simulink model "Kapitsa0x2Dpendulum"  (R2023b)
settings: Solver=VariableStepAuto  StartTime=0.0  StopTime=10  MaxStep=0.05  RelTol=1e-3
values from neighbouring files (symbols this model uses):
  Freq = freq_m(i)    [untitled.m]
  i = m*l^2    [mask1.m]
libraries: simulink_extras x2
settings Model: Creator=macbook  LastModifiedBy=macbook
settings DataIOCC: ReturnWorkspaceOutputs=off

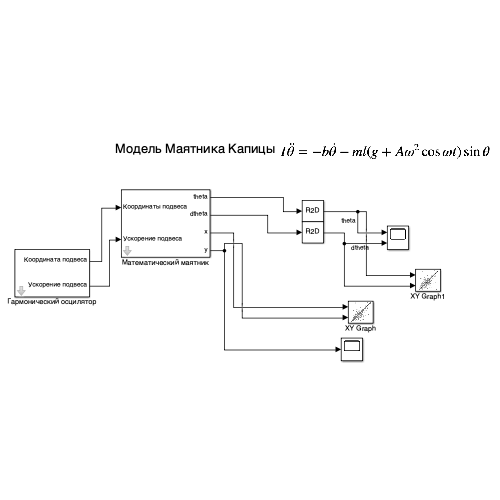
[thumbnail: Simulink's stored preview of the top-level diagram]
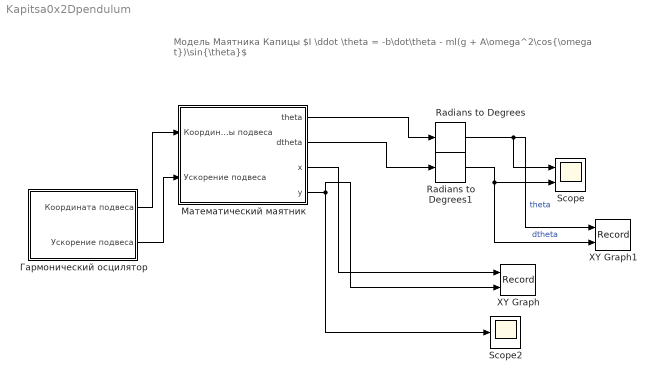
== system Kapitsa0x2Dpendulum ==
  note: Модель Маятника Капицы $I \ddot \theta = -b\dot\theta - ml(g + A\omega^2\cos{\omega t})\sin{\theta}$
  Radians to Degrees : simulink_extras/Transformations/Radians to Degrees
  Radians to Degrees1 : simulink_extras/Transformations/Radians to Degrees
  Scope : Scope  NumInputPorts=2
  Scope2 : Scope
  XY Graph : Record  FileSettingsInternal="{\"entries\":[{\"content\":{\"excelSettings\":{\"content\":{},\"type\":\"Streamout.ExcelSettings\"}},\"type\":\"Streamout.FileSettingStorage\",\"uuid\":\"\"}],\"packageUris\":[\"http:\\/\\/schema.mathworks.com\\/mf0\\/streamout_blocks\\/R2020a\"],\"version\":\"1.0\"}"  Layout=[1 1]  SignalsInternal="{\"entries\":[{\"content\":{\"signals\":[{\"content\":{\"blockPath\":[],\"dimensions\":[1],\"domain\":\"\",\"lineColor\":\"#a2142f\",\"plots\":[1],\"port\":1,\"sid\":[\"\"],\"signalID\":6339,\"signalName\":\"Математический маятник:3\"},\"type\":\"RecordBlkView.Signal\",\"uuid\":\"\"},{\"content\":{\"blockPath\":[],\"dimensions\":[1],\"domain\":\"\",\"lineColor\":\"#139fff\",\"plots\":[1],\"port\":2,\"sid\":[\"\"],\"signalID\":6343,\"signalName\":\"Математический маятник:4\"},\"type\":\"RecordBlkView.Signal\",\"uuid\":\"\"}]},\"type\":\"RecordBlkView.InputSignals\",\"uuid\":\"\"}],\"packageUris\":[\"http:\\/\\/schema.mathworks.com\\/mf0\\/streamout_blocks\\/R2020a\"],\"version\":\"1.0\"}"  VisualizationBindings="{\"xyplotplugin\":{\"info\":[{\"series\":[{\"bindingParametersList\":[{\"parameter\":\"X-Axis\",\"signalID\":6339,\"signalName\":\"Математический маятник:3\"},{\"parameter\":\"Y-Axis\",\"signalID\":6343,\"signalName\":\"Математический маятник:4\"}],\"seriesID\":5806}],\"subplotID\":1}]}}"  CompatibilityTag=XY
  XY Graph1 : Record  FileSettingsInternal="{\"entries\":[{\"content\":{\"excelSettings\":{\"content\":{},\"type\":\"Streamout.ExcelSettings\"}},\"type\":\"Streamout.FileSettingStorage\",\"uuid\":\"\"}],\"packageUris\":[\"http:\\/\\/schema.mathworks.com\\/mf0\\/streamout_blocks\\/R2020a\"],\"version\":\"1.0\"}"  Layout=[1 1]  SignalsInternal="{\"entries\":[{\"content\":{\"signals\":[{\"content\":{\"blockPath\":[],\"dimensions\":[1],\"domain\":\"\",\"lineColor\":\"#a2142f\",\"plots\":[1],\"port\":1,\"sid\":[\"\"],\"signalID\":6347,\"signalName\":\"theta\"},\"type\":\"RecordBlkView.Signal\",\"uuid\":\"\"},{\"content\":{\"blockPath\":[],\"dimensions\":[1],\"domain\":\"\",\"lineColor\":\"#139fff\",\"plots\":[1],\"port\":2,\"sid\":[\"\"],\"signalID\":6351,\"signalName\":\"dtheta\"},\"type\":\"RecordBlkView.Signal\",\"uuid\":\"\"}]},\"type\":\"RecordBlkView.InputSignals\",\"uuid\":\"\"}],\"packageUris\":[\"http:\\/\\/schema.mathworks.com\\/mf0\\/streamout_blocks\\/R2020a\"],\"version\":\"1.0\"}"  VisualizationBindings="{\"xyplotplugin\":{\"info\":[{\"series\":[{\"bindingParametersList\":[{\"parameter\":\"X-Axis\",\"signalID\":6347,\"signalName\":\"theta\"},{\"parameter\":\"Y-Axis\",\"signalID\":6351,\"signalName\":\"dtheta\"}],\"seriesID\":6880}],\"subplotID\":1}]}}"  CompatibilityTag=XY
  Гармонический осцилятор : Subsystem  mask{Ampli=0.1, Freq=Freq}
      mask prompts: Ampli "Амплитуда колебаний, м"; Freq "Частота колебаний, Гц"
  Математический маятник : Subsystem  mask{m=1, l=1, b=0.1, g=9.81, angel=120}
      mask prompts: m "Масса"; l "Длина"; angel "Начальный угол"
  wires:
  Математический маятник/1(theta) -> Radians to Degrees/1
  Математический маятник/2(dtheta) -> Radians to Degrees1/1
  Radians to Degrees/1 -> XY Graph1/1, Scope/1  "theta"
  Radians to Degrees1/1 -> XY Graph1/2, Scope/2  "dtheta"
  Математический маятник/3(x) -> XY Graph/1
  Математический маятник/4(y) -> XY Graph/2, Scope2/1
  Гармонический осцилятор/1(Координата подвеса) -> Математический маятник/1(Координаты подвеса)
  Гармонический осцилятор/2(Ускорение подвеса) -> Математический маятник/2(Ускорение подвеса)

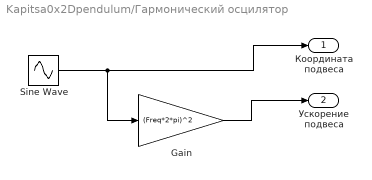
== system Kapitsa0x2Dpendulum/Гармонический осцилятор ==
  Gain : Gain  Gain=(Freq*2*pi)^2
  Sine Wave : Sin  Amplitude=Ampli  Frequency=Freq*2*pi  Phase=pi/2  SampleTime=0
  Координата подвеса : Outport
  Ускорение подвеса : Outport  Port=2
  wires:
  Sine Wave/1 -> Gain/1, Координата подвеса/1
  Gain/1 -> Ускорение подвеса/1

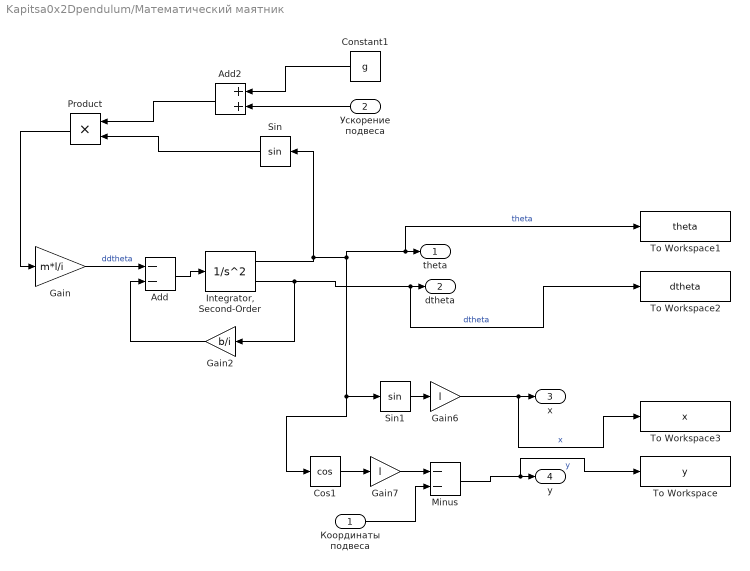
== system Kapitsa0x2Dpendulum/Математический маятник ==
  Координаты подвеса : Inport
  Ускорение подвеса : Inport  Port=2
  Add : Sum  Inputs=--
  Add2 : Sum
  Constant1 : Constant  Value=g
  Cos1 : Trigonometry  Operator=cos
  Gain : Gain  Gain=m*l/i
  Gain2 : Gain  Gain=b/i
  Gain6 : Gain  Gain=l
  Gain7 : Gain  Gain=l
  "Integrator, Second-Order" : SecondOrderIntegrator  ICX=deg2rad(angel)  ICDXDT=0
  Minus : Sum  Inputs=--
  Product : Product
  Sin : Trigonometry
  Sin1 : Trigonometry
  To Workspace : ToWorkspace  VariableName=y  SampleTime=-1
      settings: Save2DSignal=2-D array (concatenate along first dimension)
  To Workspace1 : ToWorkspace  VariableName=theta  SampleTime=-1
      settings: Save2DSignal=2-D array (concatenate along first dimension)
  To Workspace2 : ToWorkspace  VariableName=dtheta  SampleTime=-1
      settings: Save2DSignal=2-D array (concatenate along first dimension)
  To Workspace3 : ToWorkspace  VariableName=x  SampleTime=-1
      settings: Save2DSignal=2-D array (concatenate along first dimension)
  theta : Outport
  dtheta : Outport  Port=2
  x : Outport  Port=3
  y : Outport  Port=4
  wires:
  "Integrator, Second-Order"/2 -> Gain2/1, To Workspace2/1, dtheta/1  "dtheta"
  "Integrator, Second-Order"/1 -> Sin/1, To Workspace1/1, theta/1, Cos1/1, Sin1/1  "theta"
  Gain/1 -> Add/1  "ddtheta"
  Add/1 -> "Integrator, Second-Order"/1
  Gain2/1 -> Add/2
  Sin1/1 -> Gain6/1
  Gain6/1 -> To Workspace3/1, x/1  "x"
  Cos1/1 -> Gain7/1
  Minus/1 -> To Workspace/1, y/1  "y"
  Product/1 -> Gain/1
  Constant1/1 -> Add2/1
  Ускорение подвеса/1 -> Add2/2
  Add2/1 -> Product/1
  Sin/1 -> Product/2
  Gain7/1 -> Minus/1
  Координаты подвеса/1 -> Minus/2
